simulink model "sf_message_strings"  (R2025b)
settings: Solver=VariableStepAuto  StartTime=0.0  StopTime=10.0  RelTol=1e-3
settings Model: Creator=The MathWorks, Inc.  LastModifiedBy=The MathWorks, Inc.
settings SolverCC: AlgebraicLoopSolver=TrustRegion  DecoupledContinuousIntegration=on  MinimalZcImpactIntegration=on  MaxZcPerStep=1.0
settings DataIOCC: ReturnWorkspaceOutputs=off
settings OptimizationCC: ReuseModelBlockBuffer=off
settings DebuggingCC: UnconnectedInputMsg=warning  UnconnectedOutputMsg=warning  UnconnectedLineMsg=warning  ArithmeticOperatorsInVariantConditions=warning
settings ModelReferenceCC: EnableRefExpFcnMdlSchedulingChecks=on
settings SFSimCC: SimUseLocalCustomCode=off  CustomCodeUndefinedFunction=UseInterfaceOnly
settings RTWCC: RTWUseLocalCustomCode=off  GPUComputeCapability=3.5  DLArmComputeVersion=19.05

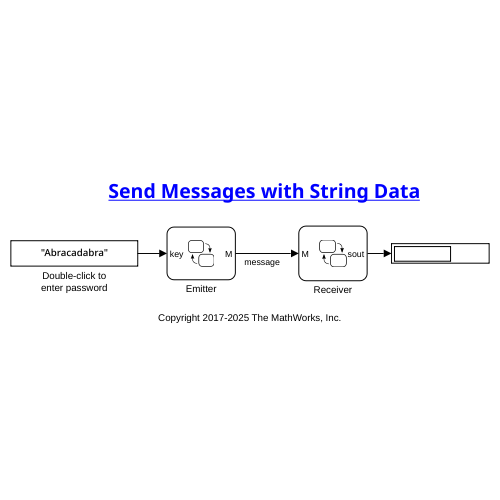
[thumbnail: Simulink's stored preview of the top-level diagram]
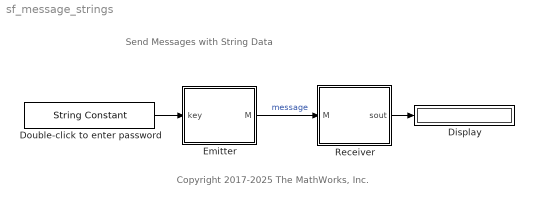
== system sf_message_strings ==
  note: Copyright 2017-2025 The MathWorks, Inc.
  note: Send Messages with String Data
  Display : Display
  Double-click to enter password : StringConstant  String="\"Abracadabra\""
  Emitter : Stateflow chart  TreatAsAtomicUnit=on
  Receiver : Stateflow chart  TreatAsAtomicUnit=on
  wires:
  Emitter/1(M) -> Receiver/1(M)  "message"
  Double-click to enter password/1 -> Emitter/1(key)
  Receiver/1(sout) -> Display/1

== stateflow chart sf_message_strings/Receiver ==
  state Off
    en,du:
    sout = 'Access Denied';
  state On
    during:
    sout = 'Access Granted';
  (default) -> Off
  Off -> On : M[M.data==lock]
  data: M input; sout output string; lock constant string ='Open Sesame'

== stateflow chart sf_message_strings/Emitter ==
  state A
    entry:
    M.data = key;
    send(M);
  (default) -> A
  data: M output string; key input
